simulink model "ldpc_encoder_580"  (R2024b)
settings: Solver=FixedStepDiscrete  StartTime=0  StopTime=0  FixedStep=1  RelTol=1e-3
model workspace (MAT data in the model file):
  G_python = [0 0 0 1 1 0 0 1 0 0 0 0 ... (668160 elements, 1152x580)]
  expected_codeword_1152 = [1 0 1 1 0 1 1 1 1 0 0 0 ... (1152 elements, 1152x1)]
  noise_mask_1152 = [0 0 0 0 0 0 0 1 0 0 0 0 ... (1152 elements, 1152x1)]
  payload_580 = [1 0 1 0 0 1 0 1 1 0 1 0 ... (580 elements, 580x1)]
(part 2 of 2)

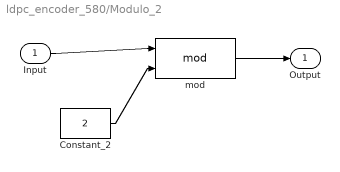
== system ldpc_encoder_580/Modulo_2 ==
  Input : Inport
  Constant_2 : Constant  Value=2
  mod : Math  Operator=mod
  Output : Outport
  wires:
  Input/1 -> mod/1
  Constant_2/1 -> mod/2
  mod/1 -> Output/1
